simulink model "bpsk_demod_architecture"  (R2023a)
settings: Solver=VariableStepAuto  StartTime=0.0  StopTime=10.0  RelTol=1e-3
settings Model: DataDictionary=bpsk_demod_interfaces.sldd  Creator=kaichiota  LastModifiedBy=kaichiota

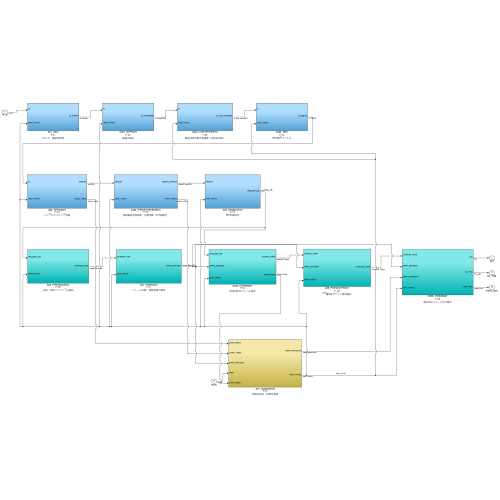
[thumbnail: Simulink's stored preview of the top-level diagram]
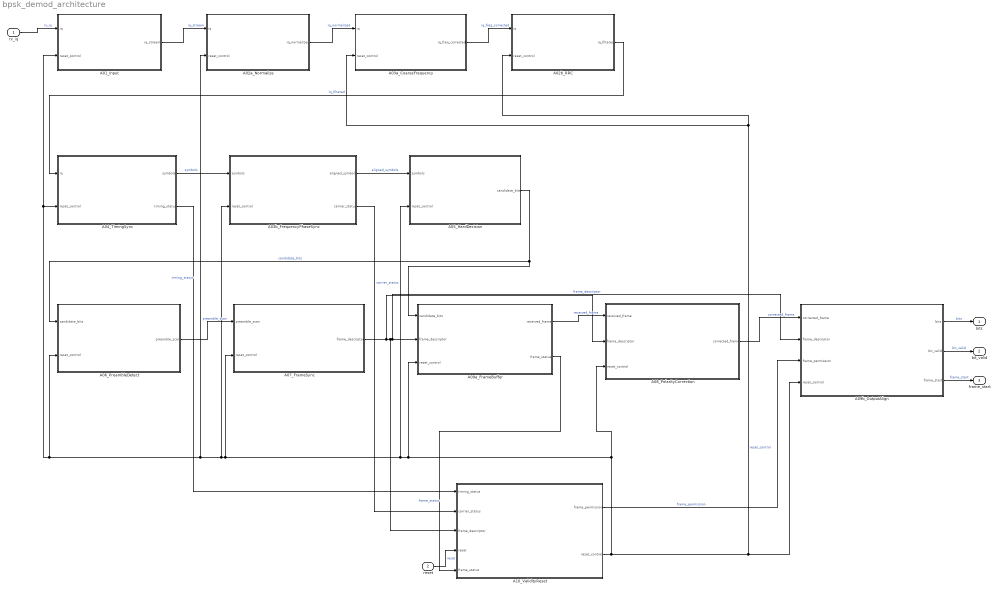
== system bpsk_demod_architecture ==
  rx_iq : Inport  Description=|  OutDataTypeStr=double  PortDimensions=1
      | IF-01 | rx_iq | complex double
      | 80 ksample/s。外部resetがfalseの間は連続入力。
      | Reset: reset中は消費しない。外部入力ポートは追加しない。
      settings: SignalType=complex
  reset : Inport  Description=|  Port=2  OutDataTypeStr=boolean  PortDimensions=1
      | IF-16 | reset | boolean
      | true中は初期化保持。
      | Reset: 外部resetを優先。bits/bit_valid/frame_startを0/false/falseへ。
  A01_Input : Subsystem  Description=|
      | F-01: IQ入力・連続性管理
      | Static architecture only. Inport/Outport placeholders; no executable algorithm. Logical signals carry position/validity metadata; data types, sizes and sample times are not specified.
      settings: AttributesFormatString=|
      | F-01
      | IQ入力・連続性管理
  A02a_Normalize : Subsystem  Description=|
      | F-02: 振幅正規化
      | Static architecture only. Inport/Outport placeholders; no executable algorithm. Logical signals carry position/validity metadata; data types, sizes and sample times are not specified.
      settings: AttributesFormatString=|
      | F-02
      | 振幅正規化
  A02b_RRC : Subsystem  Description=|
      | F-02: RRC整合フィルタ
      | Static architecture only. Inport/Outport placeholders; no executable algorithm. Logical signals carry position/validity metadata; data types, sizes and sample times are not specified.
      settings: AttributesFormatString=|
      | F-02
      | RRC整合フィルタ
  A03a_CoarseFrequency : Subsystem  Description=|
      | F-03: 搬送波周波数の粗補償（位相未同期）
      | Static architecture only. Inport/Outport placeholders; no executable algorithm. Logical signals carry position/validity metadata; data types, sizes and sample times are not specified.
      settings: AttributesFormatString=|
      | F-03
      | 搬送波周波数の粗補償（位相未同期）
  A03b_FrequencyPhaseSync : Subsystem  Description=|
      | F-03: 残留搬送波周波数・位相同期（0/π未確定）
      | Static architecture only. Inport/Outport placeholders; no executable algorithm. Logical signals carry position/validity metadata; data types, sizes and sample times are not specified.
      settings: AttributesFormatString=|
      | F-03
      | 残留搬送波周波数・位相同期（0/π未確定）
  A04_TimingSync : Subsystem  Description=|
      | F-04: シンボルタイミング同期
      | Static architecture only. Inport/Outport placeholders; no executable algorithm. Logical signals carry position/validity metadata; data types, sizes and sample times are not specified.
      settings: AttributesFormatString=|
      | F-04
      | シンボルタイミング同期
  A05_HardDecision : Subsystem  Description=|
      | F-05: BPSK硬判定
      | Static architecture only. Inport/Outport placeholders; no executable algorithm. Logical signals carry position/validity metadata; data types, sizes and sample times are not specified.
      settings: AttributesFormatString=|
      | F-05
      | BPSK硬判定
  A06_PreambleDetect : Subsystem  Description=|
      | F-06: 正規・反転プリアンブル識別
      | Static architecture only. Inport/Outport placeholders; no executable algorithm. Logical signals carry position/validity metadata; data types, sizes and sample times are not specified.
      settings: AttributesFormatString=|
      | F-06
      | 正規・反転プリアンブル識別
  A07_FrameSync : Subsystem  Description=|
      | F-07: フレーム位置・極性情報の確定
      | Static architecture only. Inport/Outport placeholders; no executable algorithm. Logical signals carry position/validity metadata; data types, sizes and sample times are not specified.
      settings: AttributesFormatString=|
      | F-07
      | フレーム位置・極性情報の確定
  A08_PolarityCorrection : Subsystem  Description=|
      | F-08: 0/π曖昧性のビット極性補正
      | Static architecture only. Inport/Outport placeholders; no executable algorithm. Logical signals carry position/validity metadata; data types, sizes and sample times are not specified.
      settings: AttributesFormatString=|
      | F-08
      | 0/π曖昧性のビット極性補正
  A09a_FrameBuffer : Subsystem  Description=|
      | F-09: 受信288 bitフレーム保持
      | Static architecture only. Inport/Outport placeholders; no executable algorithm. Logical signals carry position/validity metadata; data types, sizes and sample times are not specified.
      settings: AttributesFormatString=|
      | F-09
      | 受信288 bitフレーム保持
  A09b_OutputAlign : Subsystem  Description=|
      | F-09: 補正済みフレーム出力整列
      | Static architecture only. Inport/Outport placeholders; no executable algorithm. Logical signals carry position/validity metadata; data types, sizes and sample times are not specified.
      settings: AttributesFormatString=|
      | F-09
      | 補正済みフレーム出力整列
  A10_ValidityReset : Subsystem  Description=|
      | F-10: 同期有効性・初期化管理
      | Static architecture only. Inport/Outport placeholders; no executable algorithm. Logical signals carry position/validity metadata; data types, sizes and sample times are not specified.
      settings: AttributesFormatString=|
      | F-10
      | 同期有効性・初期化管理
  bits : Outport  Description=|  OutDataTypeStr=uint8  PortDimensions=1
      | IF-18 | bits | uint8
      | 公称10 kbit/s、bit_valid=true時のみ意味を持つ。
      | Reset: reset時0。無効区間も0。
  bit_valid : Outport  Description=|  Port=2  OutDataTypeStr=boolean  PortDimensions=1
      | IF-19 | bit_valid | boolean
      | bitsと同時。同期・位置・極性が確定した対象フレームの送出時にtrue。
      | Reset: reset時false。
  frame_start : Outport  Description=|  Port=3  OutDataTypeStr=boolean  PortDimensions=1
      | IF-20 | frame_start | boolean
      | bit_valid=trueかつフレームの最初のbitのみtrue。
      | Reset: reset時false。
  wires:
  A09b_OutputAlign/3(frame_start) -> frame_start/1  "frame_start"
  A09b_OutputAlign/2(bit_valid) -> bit_valid/1  "bit_valid"
  A09b_OutputAlign/1(bits) -> bits/1  "bits"
  A10_ValidityReset/2(reset_control) -> A03a_CoarseFrequency/2(reset_control), A02b_RRC/2(reset_control), A09b_OutputAlign/4(reset_control), A01_Input/2(reset_control), A04_TimingSync/2(reset_control), A06_PreambleDetect/2(reset_control), A02a_Normalize/2(reset_control), A03b_FrequencyPhaseSync/2(reset_control), A07_FrameSync/2(reset_control), A05_HardDecision/2(reset_control), A09a_FrameBuffer/3(reset_control), A08_PolarityCorrection/3(reset_control)  "reset_control"
  reset/1 -> A10_ValidityReset/4(reset)  "reset"
  A10_ValidityReset/1(frame_permission) -> A09b_OutputAlign/3(frame_permission)  "frame_permission"
  A03b_FrequencyPhaseSync/2(carrier_status) -> A10_ValidityReset/2(carrier_status)  "carrier_status"
  A04_TimingSync/2(timing_status) -> A10_ValidityReset/1(timing_status)  "timing_status"
  A08_PolarityCorrection/1(corrected_frame) -> A09b_OutputAlign/1(corrected_frame)  "corrected_frame"
  A09a_FrameBuffer/1(received_frame) -> A08_PolarityCorrection/1(received_frame)  "received_frame"
  A07_FrameSync/1(frame_descriptor) -> A09b_OutputAlign/2(frame_descriptor), A09a_FrameBuffer/2(frame_descriptor), A10_ValidityReset/3(frame_descriptor), A08_PolarityCorrection/2(frame_descriptor)  "frame_descriptor"
  A06_PreambleDetect/1(preamble_scan) -> A07_FrameSync/1(preamble_scan)  "preamble_scan"
  A05_HardDecision/1(candidate_bits) -> A09a_FrameBuffer/1(candidate_bits), A06_PreambleDetect/1(candidate_bits)  "candidate_bits"
  A03b_FrequencyPhaseSync/1(aligned_symbols) -> A05_HardDecision/1(symbols)  "aligned_symbols"
  A04_TimingSync/1(symbols) -> A03b_FrequencyPhaseSync/1(symbols)  "symbols"
  A02b_RRC/1(iq_filtered) -> A04_TimingSync/1(iq)  "iq_filtered"
  A03a_CoarseFrequency/1(iq_freq_corrected) -> A02b_RRC/1(iq)  "iq_freq_corrected"
  A02a_Normalize/1(iq_normalized) -> A03a_CoarseFrequency/1(iq)  "iq_normalized"
  A01_Input/1(iq_stream) -> A02a_Normalize/1(iq)  "iq_stream"
  rx_iq/1 -> A01_Input/1(iq)  "rx_iq"
  A09a_FrameBuffer/2(frame_status) -> A10_ValidityReset/5(frame_status)  "frame_status"

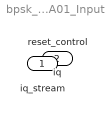
== system bpsk_demod_architecture/A01_Input ==
  iq : Inport  Description=|  OutDataTypeStr=double  PortDimensions=1
      | IF-01 | rx_iq | complex double
      | 80 ksample/s。外部resetがfalseの間は連続入力。
      | Reset: reset中は消費しない。外部入力ポートは追加しない。
      settings: SignalType=complex
  reset_control : Inport  Description=|  Port=2  OutDataTypeStr=Bus: ResetControl
      | IF-17 | reset_control | ResetControl
      | データより先に適用。resetは全初期化、epoch更新のみは再捕捉。
      | Reset: 外部reset区間の開始または再捕捉要求ごとにepochを1回更新。reset保持中は維持。再捕捉時はA-09b受理済みの許可済み完成フレームを保持し、外部resetでは全破棄。
      | reset: boolean scalar — trueの間は保持状態・出力有効を初期化し新規データを消費しない。
      | epoch: uint64 scalar — 実行開始は0。外部reset区間の開始または再捕捉要求ごとに更新し、reset保持中は維持。reset=falseでの更新は再捕捉。旧epochの未許可情報を破棄し、A-09bで受理済みの許可済み完成フレームだけ送出を継続する。
  iq_stream : Outport  Description=|  OutDataTypeStr=Bus: IqRecord
      | IF-02 | iq_stream | IqRecord
      | 80 ksample/s、valid時のみ消費。
      | Reset: 初期化時はvalid=false、旧epochの情報を破棄。
      | valid: boolean scalar — 新しいレコードがある場合true。false時は他フィールドを消費しない。
      | epoch: uint64 scalar — 初期化区間のID。異なるepochのデータ・制御を結合しない。
      | sample_index: uint64 scalar — A-01が付与する0始まり入力サンプル位置。80 ksample/s処理間で維持。
      | value: complex double scalar — 受信または処理後IQ。
      | usable: boolean scalar — 後続の同期判定への利用可否。A-03aは入力の利用可否と粗周波数推定の利用可否を反映し、A-02bはフィルタ過渡も加味する。falseは後段でtrueに上書きしない。具体判定条件は次工程。

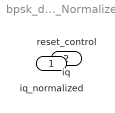
== system bpsk_demod_architecture/A02a_Normalize ==
  iq : Inport  Description=|  OutDataTypeStr=Bus: IqRecord
      | IF-02 | iq_stream | IqRecord
      | 80 ksample/s、valid時のみ消費。
      | Reset: 初期化時はvalid=false、旧epochの情報を破棄。
      | valid: boolean scalar — 新しいレコードがある場合true。false時は他フィールドを消費しない。
      | epoch: uint64 scalar — 初期化区間のID。異なるepochのデータ・制御を結合しない。
      | sample_index: uint64 scalar — A-01が付与する0始まり入力サンプル位置。80 ksample/s処理間で維持。
      | value: complex double scalar — 受信または処理後IQ。
      | usable: boolean scalar — 後続の同期判定への利用可否。A-03aは入力の利用可否と粗周波数推定の利用可否を反映し、A-02bはフィルタ過渡も加味する。falseは後段でtrueに上書きしない。具体判定条件は次工程。
  reset_control : Inport  Description=|  Port=2  OutDataTypeStr=Bus: ResetControl
      | IF-17 | reset_control | ResetControl
      | データより先に適用。resetは全初期化、epoch更新のみは再捕捉。
      | Reset: 外部reset区間の開始または再捕捉要求ごとにepochを1回更新。reset保持中は維持。再捕捉時はA-09b受理済みの許可済み完成フレームを保持し、外部resetでは全破棄。
      | reset: boolean scalar — trueの間は保持状態・出力有効を初期化し新規データを消費しない。
      | epoch: uint64 scalar — 実行開始は0。外部reset区間の開始または再捕捉要求ごとに更新し、reset保持中は維持。reset=falseでの更新は再捕捉。旧epochの未許可情報を破棄し、A-09bで受理済みの許可済み完成フレームだけ送出を継続する。
  iq_normalized : Outport  Description=|  OutDataTypeStr=Bus: IqRecord
      | IF-03 | iq_normalized | IqRecord
      | 80 ksample/s、valid時のみ消費。
      | Reset: 初期化時はvalid=false、旧epochの情報を破棄。
      | valid: boolean scalar — 新しいレコードがある場合true。false時は他フィールドを消費しない。
      | epoch: uint64 scalar — 初期化区間のID。異なるepochのデータ・制御を結合しない。
      | sample_index: uint64 scalar — A-01が付与する0始まり入力サンプル位置。80 ksample/s処理間で維持。
      | value: complex double scalar — 受信または処理後IQ。
      | usable: boolean scalar — 後続の同期判定への利用可否。A-03aは入力の利用可否と粗周波数推定の利用可否を反映し、A-02bはフィルタ過渡も加味する。falseは後段でtrueに上書きしない。具体判定条件は次工程。

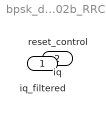
== system bpsk_demod_architecture/A02b_RRC ==
  iq : Inport  Description=|  OutDataTypeStr=Bus: IqRecord
      | IF-04 | iq_freq_corrected | IqRecord
      | 80 ksample/s、valid時のみ消費。
      | Reset: 初期化時はvalid=false、旧epochの情報を破棄。
      | valid: boolean scalar — 新しいレコードがある場合true。false時は他フィールドを消費しない。
      | epoch: uint64 scalar — 初期化区間のID。異なるepochのデータ・制御を結合しない。
      | sample_index: uint64 scalar — A-01が付与する0始まり入力サンプル位置。80 ksample/s処理間で維持。
      | value: complex double scalar — 受信または処理後IQ。
      | usable: boolean scalar — 後続の同期判定への利用可否。A-03aは入力の利用可否と粗周波数推定の利用可否を反映し、A-02bはフィルタ過渡も加味する。falseは後段でtrueに上書きしない。具体判定条件は次工程。
  reset_control : Inport  Description=|  Port=2  OutDataTypeStr=Bus: ResetControl
      | IF-17 | reset_control | ResetControl
      | データより先に適用。resetは全初期化、epoch更新のみは再捕捉。
      | Reset: 外部reset区間の開始または再捕捉要求ごとにepochを1回更新。reset保持中は維持。再捕捉時はA-09b受理済みの許可済み完成フレームを保持し、外部resetでは全破棄。
      | reset: boolean scalar — trueの間は保持状態・出力有効を初期化し新規データを消費しない。
      | epoch: uint64 scalar — 実行開始は0。外部reset区間の開始または再捕捉要求ごとに更新し、reset保持中は維持。reset=falseでの更新は再捕捉。旧epochの未許可情報を破棄し、A-09bで受理済みの許可済み完成フレームだけ送出を継続する。
  iq_filtered : Outport  Description=|  OutDataTypeStr=Bus: IqRecord
      | IF-05 | iq_filtered | IqRecord
      | 80 ksample/s、valid時のみ消費。
      | Reset: 初期化時はvalid=false、旧epochの情報を破棄。
      | valid: boolean scalar — 新しいレコードがある場合true。false時は他フィールドを消費しない。
      | epoch: uint64 scalar — 初期化区間のID。異なるepochのデータ・制御を結合しない。
      | sample_index: uint64 scalar — A-01が付与する0始まり入力サンプル位置。80 ksample/s処理間で維持。
      | value: complex double scalar — 受信または処理後IQ。
      | usable: boolean scalar — 後続の同期判定への利用可否。A-03aは入力の利用可否と粗周波数推定の利用可否を反映し、A-02bはフィルタ過渡も加味する。falseは後段でtrueに上書きしない。具体判定条件は次工程。

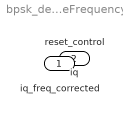
== system bpsk_demod_architecture/A03a_CoarseFrequency ==
  iq : Inport  Description=|  OutDataTypeStr=Bus: IqRecord
      | IF-03 | iq_normalized | IqRecord
      | 80 ksample/s、valid時のみ消費。
      | Reset: 初期化時はvalid=false、旧epochの情報を破棄。
      | valid: boolean scalar — 新しいレコードがある場合true。false時は他フィールドを消費しない。
      | epoch: uint64 scalar — 初期化区間のID。異なるepochのデータ・制御を結合しない。
      | sample_index: uint64 scalar — A-01が付与する0始まり入力サンプル位置。80 ksample/s処理間で維持。
      | value: complex double scalar — 受信または処理後IQ。
      | usable: boolean scalar — 後続の同期判定への利用可否。A-03aは入力の利用可否と粗周波数推定の利用可否を反映し、A-02bはフィルタ過渡も加味する。falseは後段でtrueに上書きしない。具体判定条件は次工程。
  reset_control : Inport  Description=|  Port=2  OutDataTypeStr=Bus: ResetControl
      | IF-17 | reset_control | ResetControl
      | データより先に適用。resetは全初期化、epoch更新のみは再捕捉。
      | Reset: 外部reset区間の開始または再捕捉要求ごとにepochを1回更新。reset保持中は維持。再捕捉時はA-09b受理済みの許可済み完成フレームを保持し、外部resetでは全破棄。
      | reset: boolean scalar — trueの間は保持状態・出力有効を初期化し新規データを消費しない。
      | epoch: uint64 scalar — 実行開始は0。外部reset区間の開始または再捕捉要求ごとに更新し、reset保持中は維持。reset=falseでの更新は再捕捉。旧epochの未許可情報を破棄し、A-09bで受理済みの許可済み完成フレームだけ送出を継続する。
  iq_freq_corrected : Outport  Description=|  OutDataTypeStr=Bus: IqRecord
      | IF-04 | iq_freq_corrected | IqRecord
      | 80 ksample/s、valid時のみ消費。
      | Reset: 初期化時はvalid=false、旧epochの情報を破棄。
      | valid: boolean scalar — 新しいレコードがある場合true。false時は他フィールドを消費しない。
      | epoch: uint64 scalar — 初期化区間のID。異なるepochのデータ・制御を結合しない。
      | sample_index: uint64 scalar — A-01が付与する0始まり入力サンプル位置。80 ksample/s処理間で維持。
      | value: complex double scalar — 受信または処理後IQ。
      | usable: boolean scalar — 後続の同期判定への利用可否。A-03aは入力の利用可否と粗周波数推定の利用可否を反映し、A-02bはフィルタ過渡も加味する。falseは後段でtrueに上書きしない。具体判定条件は次工程。

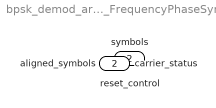
== system bpsk_demod_architecture/A03b_FrequencyPhaseSync ==
  symbols : Inport  Description=|  OutDataTypeStr=Bus: SymbolRecord
      | IF-06 | symbols | SymbolRecord
      | 公称10 ksymbol/s。validな候補ごとに更新。
      | Reset: 初期化時はvalid=false、旧epochの情報を破棄。
      | valid: boolean scalar — 新しいレコードがある場合true。false時は他フィールドを消費しない。
      | epoch: uint64 scalar — 初期化区間のID。異なるepochのデータ・制御を結合しない。
      | symbol_index: uint64 scalar — A-04が候補シンボル生成順に0から付与。同期未確立でも生成した候補は数える。
      | value: complex double scalar — 抽出または搬送波補償後のシンボル。
      | timing_locked: boolean scalar — 当該シンボルに対応するタイミング同期状態。入力usableも加味する。
      | carrier_locked: boolean scalar — 当該シンボルの搬送波同期状態。A-04ではfalse、A-03bが設定。
  reset_control : Inport  Description=|  Port=2  OutDataTypeStr=Bus: ResetControl
      | IF-17 | reset_control | ResetControl
      | データより先に適用。resetは全初期化、epoch更新のみは再捕捉。
      | Reset: 外部reset区間の開始または再捕捉要求ごとにepochを1回更新。reset保持中は維持。再捕捉時はA-09b受理済みの許可済み完成フレームを保持し、外部resetでは全破棄。
      | reset: boolean scalar — trueの間は保持状態・出力有効を初期化し新規データを消費しない。
      | epoch: uint64 scalar — 実行開始は0。外部reset区間の開始または再捕捉要求ごとに更新し、reset保持中は維持。reset=falseでの更新は再捕捉。旧epochの未許可情報を破棄し、A-09bで受理済みの許可済み完成フレームだけ送出を継続する。
  aligned_symbols : Outport  Description=|  OutDataTypeStr=Bus: SymbolRecord
      | IF-07 | aligned_symbols | SymbolRecord
      | IF-06の位置を保持。
      | Reset: 初期化時はvalid=false、旧epochの情報を破棄。
      | valid: boolean scalar — 新しいレコードがある場合true。false時は他フィールドを消費しない。
      | epoch: uint64 scalar — 初期化区間のID。異なるepochのデータ・制御を結合しない。
      | symbol_index: uint64 scalar — A-04が候補シンボル生成順に0から付与。同期未確立でも生成した候補は数える。
      | value: complex double scalar — 抽出または搬送波補償後のシンボル。
      | timing_locked: boolean scalar — 当該シンボルに対応するタイミング同期状態。入力usableも加味する。
      | carrier_locked: boolean scalar — 当該シンボルの搬送波同期状態。A-04ではfalse、A-03bが設定。
  carrier_status : Outport  Description=|  Port=2  OutDataTypeStr=Bus: SyncStatus
      | IF-14 | carrier_status | SyncStatus
      | 候補シンボルごとの搬送波同期状態。
      | Reset: 初期化時はvalid=false、旧epochの情報を破棄。
      | valid: boolean scalar — 新しいレコードがある場合true。false時は他フィールドを消費しない。
      | epoch: uint64 scalar — 初期化区間のID。異なるepochのデータ・制御を結合しない。
      | symbol_index: uint64 scalar — この同期判定が対応する候補シンボル位置。
      | locked: boolean scalar — タイミングまたは搬送波の同期成立判定。具体閾値・継続条件は次工程。

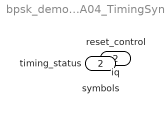
== system bpsk_demod_architecture/A04_TimingSync ==
  iq : Inport  Description=|  OutDataTypeStr=Bus: IqRecord
      | IF-05 | iq_filtered | IqRecord
      | 80 ksample/s、valid時のみ消費。
      | Reset: 初期化時はvalid=false、旧epochの情報を破棄。
      | valid: boolean scalar — 新しいレコードがある場合true。false時は他フィールドを消費しない。
      | epoch: uint64 scalar — 初期化区間のID。異なるepochのデータ・制御を結合しない。
      | sample_index: uint64 scalar — A-01が付与する0始まり入力サンプル位置。80 ksample/s処理間で維持。
      | value: complex double scalar — 受信または処理後IQ。
      | usable: boolean scalar — 後続の同期判定への利用可否。A-03aは入力の利用可否と粗周波数推定の利用可否を反映し、A-02bはフィルタ過渡も加味する。falseは後段でtrueに上書きしない。具体判定条件は次工程。
  reset_control : Inport  Description=|  Port=2  OutDataTypeStr=Bus: ResetControl
      | IF-17 | reset_control | ResetControl
      | データより先に適用。resetは全初期化、epoch更新のみは再捕捉。
      | Reset: 外部reset区間の開始または再捕捉要求ごとにepochを1回更新。reset保持中は維持。再捕捉時はA-09b受理済みの許可済み完成フレームを保持し、外部resetでは全破棄。
      | reset: boolean scalar — trueの間は保持状態・出力有効を初期化し新規データを消費しない。
      | epoch: uint64 scalar — 実行開始は0。外部reset区間の開始または再捕捉要求ごとに更新し、reset保持中は維持。reset=falseでの更新は再捕捉。旧epochの未許可情報を破棄し、A-09bで受理済みの許可済み完成フレームだけ送出を継続する。
  symbols : Outport  Description=|  OutDataTypeStr=Bus: SymbolRecord
      | IF-06 | symbols | SymbolRecord
      | 公称10 ksymbol/s。validな候補ごとに更新。
      | Reset: 初期化時はvalid=false、旧epochの情報を破棄。
      | valid: boolean scalar — 新しいレコードがある場合true。false時は他フィールドを消費しない。
      | epoch: uint64 scalar — 初期化区間のID。異なるepochのデータ・制御を結合しない。
      | symbol_index: uint64 scalar — A-04が候補シンボル生成順に0から付与。同期未確立でも生成した候補は数える。
      | value: complex double scalar — 抽出または搬送波補償後のシンボル。
      | timing_locked: boolean scalar — 当該シンボルに対応するタイミング同期状態。入力usableも加味する。
      | carrier_locked: boolean scalar — 当該シンボルの搬送波同期状態。A-04ではfalse、A-03bが設定。
  timing_status : Outport  Description=|  Port=2  OutDataTypeStr=Bus: SyncStatus
      | IF-13 | timing_status | SyncStatus
      | 候補シンボルごとのタイミング同期状態。
      | Reset: 初期化時はvalid=false、旧epochの情報を破棄。
      | valid: boolean scalar — 新しいレコードがある場合true。false時は他フィールドを消費しない。
      | epoch: uint64 scalar — 初期化区間のID。異なるepochのデータ・制御を結合しない。
      | symbol_index: uint64 scalar — この同期判定が対応する候補シンボル位置。
      | locked: boolean scalar — タイミングまたは搬送波の同期成立判定。具体閾値・継続条件は次工程。

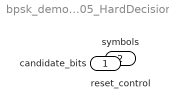
== system bpsk_demod_architecture/A05_HardDecision ==
  symbols : Inport  Description=|  OutDataTypeStr=Bus: SymbolRecord
      | IF-07 | aligned_symbols | SymbolRecord
      | IF-06の位置を保持。
      | Reset: 初期化時はvalid=false、旧epochの情報を破棄。
      | valid: boolean scalar — 新しいレコードがある場合true。false時は他フィールドを消費しない。
      | epoch: uint64 scalar — 初期化区間のID。異なるepochのデータ・制御を結合しない。
      | symbol_index: uint64 scalar — A-04が候補シンボル生成順に0から付与。同期未確立でも生成した候補は数える。
      | value: complex double scalar — 抽出または搬送波補償後のシンボル。
      | timing_locked: boolean scalar — 当該シンボルに対応するタイミング同期状態。入力usableも加味する。
      | carrier_locked: boolean scalar — 当該シンボルの搬送波同期状態。A-04ではfalse、A-03bが設定。
  reset_control : Inport  Description=|  Port=2  OutDataTypeStr=Bus: ResetControl
      | IF-17 | reset_control | ResetControl
      | データより先に適用。resetは全初期化、epoch更新のみは再捕捉。
      | Reset: 外部reset区間の開始または再捕捉要求ごとにepochを1回更新。reset保持中は維持。再捕捉時はA-09b受理済みの許可済み完成フレームを保持し、外部resetでは全破棄。
      | reset: boolean scalar — trueの間は保持状態・出力有効を初期化し新規データを消費しない。
      | epoch: uint64 scalar — 実行開始は0。外部reset区間の開始または再捕捉要求ごとに更新し、reset保持中は維持。reset=falseでの更新は再捕捉。旧epochの未許可情報を破棄し、A-09bで受理済みの許可済み完成フレームだけ送出を継続する。
  candidate_bits : Outport  Description=|  OutDataTypeStr=Bus: BitRecord
      | IF-08 | candidate_bits | BitRecord
      | 公称10 kbit/s。validとsync_okを区別。
      | Reset: 初期化時はvalid=false、旧epochの情報を破棄。
      | valid: boolean scalar — 新しいレコードがある場合true。false時は他フィールドを消費しない。
      | epoch: uint64 scalar — 初期化区間のID。異なるepochのデータ・制御を結合しない。
      | bit_index: uint64 scalar — 対応するsymbol_indexをそのまま継承。候補bitの0始まり位置。
      | value: uint8 scalar — 極性未確定の硬判定0/1。
      | sync_ok: boolean scalar — 当該シンボルのtiming_locked AND carrier_locked。falseでもvalidな候補は位置を進める。

== system bpsk_demod_architecture/A06_PreambleDetect ==
  candidate_bits : Inport  Description=|  OutDataTypeStr=Bus: BitRecord
      | IF-08 | candidate_bits | BitRecord
      | 公称10 kbit/s。validとsync_okを区別。
      | Reset: 初期化時はvalid=false、旧epochの情報を破棄。
      | valid: boolean scalar — 新しいレコードがある場合true。false時は他フィールドを消費しない。
      | epoch: uint64 scalar — 初期化区間のID。異なるepochのデータ・制御を結合しない。
      | bit_index: uint64 scalar — 対応するsymbol_indexをそのまま継承。候補bitの0始まり位置。
      | value: uint8 scalar — 極性未確定の硬判定0/1。
      | sync_ok: boolean scalar — 当該シンボルのtiming_locked AND carrier_locked。falseでもvalidな候補は位置を進める。
  reset_control : Inport  Description=|  Port=2  OutDataTypeStr=Bus: ResetControl
      | IF-17 | reset_control | ResetControl
      | データより先に適用。resetは全初期化、epoch更新のみは再捕捉。
      | Reset: 外部reset区間の開始または再捕捉要求ごとにepochを1回更新。reset保持中は維持。再捕捉時はA-09b受理済みの許可済み完成フレームを保持し、外部resetでは全破棄。
      | reset: boolean scalar — trueの間は保持状態・出力有効を初期化し新規データを消費しない。
      | epoch: uint64 scalar — 実行開始は0。外部reset区間の開始または再捕捉要求ごとに更新し、reset保持中は維持。reset=falseでの更新は再捕捉。旧epochの未許可情報を破棄し、A-09bで受理済みの許可済み完成フレームだけ送出を継続する。
  preamble_scan : Outport  Description=|  OutDataTypeStr=Bus: PreambleScan
      | IF-09 | preamble_scan | PreambleScan
      | 候補bitごと。未検出時もvalid=trueで進捗を通知。
      | Reset: 初期化時はvalid=false、旧epochの情報を破棄。
      | valid: boolean scalar — 新しいレコードがある場合true。false時は他フィールドを消費しない。
      | epoch: uint64 scalar — 初期化区間のID。異なるepochのデータ・制御を結合しない。
      | bit_index: uint64 scalar — 照合窓末尾の候補bit位置。未検出時も通知し、A-07が期待位置を通過したことを認識できる。
      | window_ready: boolean scalar — 連続した32 bitの窓が揃ったか。
      | match_found: boolean scalar — 正規または反転パターンの候補として採用可能か。閾値・同点処理は未定。
      | start_bit: uint64 scalar — window_ready時のみ有効。bit_index-31。
      | invert: boolean scalar — match_found時のみ有効。trueなら全bit反転候補。
      | errors_normal: uint8 scalar — window_ready時の正規プリアンブルとの不一致数0〜32。
      | errors_inverted: uint8 scalar — window_ready時の反転プリアンブルとの不一致数0〜32。
      | window_sync_ok: boolean scalar — 照合対象32 bitすべてでsync_okがtrueか。

== system bpsk_demod_architecture/A07_FrameSync ==
  preamble_scan : Inport  Description=|  OutDataTypeStr=Bus: PreambleScan
      | IF-09 | preamble_scan | PreambleScan
      | 候補bitごと。未検出時もvalid=trueで進捗を通知。
      | Reset: 初期化時はvalid=false、旧epochの情報を破棄。
      | valid: boolean scalar — 新しいレコードがある場合true。false時は他フィールドを消費しない。
      | epoch: uint64 scalar — 初期化区間のID。異なるepochのデータ・制御を結合しない。
      | bit_index: uint64 scalar — 照合窓末尾の候補bit位置。未検出時も通知し、A-07が期待位置を通過したことを認識できる。
      | window_ready: boolean scalar — 連続した32 bitの窓が揃ったか。
      | match_found: boolean scalar — 正規または反転パターンの候補として採用可能か。閾値・同点処理は未定。
      | start_bit: uint64 scalar — window_ready時のみ有効。bit_index-31。
      | invert: boolean scalar — match_found時のみ有効。trueなら全bit反転候補。
      | errors_normal: uint8 scalar — window_ready時の正規プリアンブルとの不一致数0〜32。
      | errors_inverted: uint8 scalar — window_ready時の反転プリアンブルとの不一致数0〜32。
      | window_sync_ok: boolean scalar — 照合対象32 bitすべてでsync_okがtrueか。
  reset_control : Inport  Description=|  Port=2  OutDataTypeStr=Bus: ResetControl
      | IF-17 | reset_control | ResetControl
      | データより先に適用。resetは全初期化、epoch更新のみは再捕捉。
      | Reset: 外部reset区間の開始または再捕捉要求ごとにepochを1回更新。reset保持中は維持。再捕捉時はA-09b受理済みの許可済み完成フレームを保持し、外部resetでは全破棄。
      | reset: boolean scalar — trueの間は保持状態・出力有効を初期化し新規データを消費しない。
      | epoch: uint64 scalar — 実行開始は0。外部reset区間の開始または再捕捉要求ごとに更新し、reset保持中は維持。reset=falseでの更新は再捕捉。旧epochの未許可情報を破棄し、A-09bで受理済みの許可済み完成フレームだけ送出を継続する。
  frame_descriptor : Outport  Description=|  OutDataTypeStr=Bus: FrameDescriptor
      | IF-10 | frame_descriptor | FrameDescriptor
      | フレーム判断イベント。位置・極性が揃うまでconfirmed=false。
      | Reset: 初期化時はvalid=false、旧epochの情報を破棄。
      | valid: boolean scalar — 新しいレコードがある場合true。false時は他フィールドを消費しない。
      | epoch: uint64 scalar — 初期化区間のID。異なるepochのデータ・制御を結合しない。
      | start_bit: uint64 scalar — 対象フレームのプリアンブル先頭bit位置。epochと合わせてフレームキーとする。
      | confirmed: boolean scalar — 当該フレームの位置とプリアンブルが確認済みか。未検出等ではfalse。
      | polarity_valid: boolean scalar — invertが有効な極性判断か。
      | invert: boolean scalar — trueなら対象288 bitを反転。polarity_valid=falseのとき解釈しない。

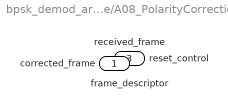
== system bpsk_demod_architecture/A08_PolarityCorrection ==
  received_frame : Inport  Description=|  OutDataTypeStr=Bus: ReceivedFrame
      | IF-11 | received_frame | ReceivedFrame
      | 完成フレームごと。未完成のbit配列は出さない。
      | Reset: 初期化時はvalid=false、旧epochの情報を破棄。
      | valid: boolean scalar — 新しいレコードがある場合true。false時は他フィールドを消費しない。
      | epoch: uint64 scalar — 初期化区間のID。異なるepochのデータ・制御を結合しない。
      | start_bit: uint64 scalar — 保持フレームの先頭。
      | bits: uint8 [288,1] — 受信順の0/1。先頭32要素がプリアンブル、残り256要素がデータ。
      | sync_ok_all: boolean scalar — 対象288 bitのsync_okの論理積。現在のロック状態で代用しない。
  frame_descriptor : Inport  Description=|  Port=2  OutDataTypeStr=Bus: FrameDescriptor
      | IF-10 | frame_descriptor | FrameDescriptor
      | フレーム判断イベント。位置・極性が揃うまでconfirmed=false。
      | Reset: 初期化時はvalid=false、旧epochの情報を破棄。
      | valid: boolean scalar — 新しいレコードがある場合true。false時は他フィールドを消費しない。
      | epoch: uint64 scalar — 初期化区間のID。異なるepochのデータ・制御を結合しない。
      | start_bit: uint64 scalar — 対象フレームのプリアンブル先頭bit位置。epochと合わせてフレームキーとする。
      | confirmed: boolean scalar — 当該フレームの位置とプリアンブルが確認済みか。未検出等ではfalse。
      | polarity_valid: boolean scalar — invertが有効な極性判断か。
      | invert: boolean scalar — trueなら対象288 bitを反転。polarity_valid=falseのとき解釈しない。
  reset_control : Inport  Description=|  Port=3  OutDataTypeStr=Bus: ResetControl
      | IF-17 | reset_control | ResetControl
      | データより先に適用。resetは全初期化、epoch更新のみは再捕捉。
      | Reset: 外部reset区間の開始または再捕捉要求ごとにepochを1回更新。reset保持中は維持。再捕捉時はA-09b受理済みの許可済み完成フレームを保持し、外部resetでは全破棄。
      | reset: boolean scalar — trueの間は保持状態・出力有効を初期化し新規データを消費しない。
      | epoch: uint64 scalar — 実行開始は0。外部reset区間の開始または再捕捉要求ごとに更新し、reset保持中は維持。reset=falseでの更新は再捕捉。旧epochの未許可情報を破棄し、A-09bで受理済みの許可済み完成フレームだけ送出を継続する。
  corrected_frame : Outport  Description=|  OutDataTypeStr=Bus: CorrectedFrame
      | IF-12 | corrected_frame | CorrectedFrame
      | 同一キーのReceivedFrameと有効なFrameDescriptorが揃ったとき。
      | Reset: 初期化時はvalid=false、旧epochの情報を破棄。
      | valid: boolean scalar — 新しいレコードがある場合true。false時は他フィールドを消費しない。
      | epoch: uint64 scalar — 初期化区間のID。異なるepochのデータ・制御を結合しない。
      | start_bit: uint64 scalar — 元の受信フレームと同じ先頭。
      | bits: uint8 [288,1] — 極性補正済み0/1。受信プリアンブルも同じ規則で補正し置換しない。
      | sync_ok_all: boolean scalar — ReceivedFrameから継承する。
      | inverted: boolean scalar — 実際に全bit反転を適用したか。

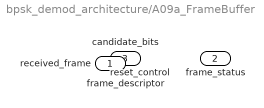
== system bpsk_demod_architecture/A09a_FrameBuffer ==
  candidate_bits : Inport  Description=|  OutDataTypeStr=Bus: BitRecord
      | IF-08 | candidate_bits | BitRecord
      | 公称10 kbit/s。validとsync_okを区別。
      | Reset: 初期化時はvalid=false、旧epochの情報を破棄。
      | valid: boolean scalar — 新しいレコードがある場合true。false時は他フィールドを消費しない。
      | epoch: uint64 scalar — 初期化区間のID。異なるepochのデータ・制御を結合しない。
      | bit_index: uint64 scalar — 対応するsymbol_indexをそのまま継承。候補bitの0始まり位置。
      | value: uint8 scalar — 極性未確定の硬判定0/1。
      | sync_ok: boolean scalar — 当該シンボルのtiming_locked AND carrier_locked。falseでもvalidな候補は位置を進める。
  frame_descriptor : Inport  Description=|  Port=2  OutDataTypeStr=Bus: FrameDescriptor
      | IF-10 | frame_descriptor | FrameDescriptor
      | フレーム判断イベント。位置・極性が揃うまでconfirmed=false。
      | Reset: 初期化時はvalid=false、旧epochの情報を破棄。
      | valid: boolean scalar — 新しいレコードがある場合true。false時は他フィールドを消費しない。
      | epoch: uint64 scalar — 初期化区間のID。異なるepochのデータ・制御を結合しない。
      | start_bit: uint64 scalar — 対象フレームのプリアンブル先頭bit位置。epochと合わせてフレームキーとする。
      | confirmed: boolean scalar — 当該フレームの位置とプリアンブルが確認済みか。未検出等ではfalse。
      | polarity_valid: boolean scalar — invertが有効な極性判断か。
      | invert: boolean scalar — trueなら対象288 bitを反転。polarity_valid=falseのとき解釈しない。
  reset_control : Inport  Description=|  Port=3  OutDataTypeStr=Bus: ResetControl
      | IF-17 | reset_control | ResetControl
      | データより先に適用。resetは全初期化、epoch更新のみは再捕捉。
      | Reset: 外部reset区間の開始または再捕捉要求ごとにepochを1回更新。reset保持中は維持。再捕捉時はA-09b受理済みの許可済み完成フレームを保持し、外部resetでは全破棄。
      | reset: boolean scalar — trueの間は保持状態・出力有効を初期化し新規データを消費しない。
      | epoch: uint64 scalar — 実行開始は0。外部reset区間の開始または再捕捉要求ごとに更新し、reset保持中は維持。reset=falseでの更新は再捕捉。旧epochの未許可情報を破棄し、A-09bで受理済みの許可済み完成フレームだけ送出を継続する。
  received_frame : Outport  Description=|  OutDataTypeStr=Bus: ReceivedFrame
      | IF-11 | received_frame | ReceivedFrame
      | 完成フレームごと。未完成のbit配列は出さない。
      | Reset: 初期化時はvalid=false、旧epochの情報を破棄。
      | valid: boolean scalar — 新しいレコードがある場合true。false時は他フィールドを消費しない。
      | epoch: uint64 scalar — 初期化区間のID。異なるepochのデータ・制御を結合しない。
      | start_bit: uint64 scalar — 保持フレームの先頭。
      | bits: uint8 [288,1] — 受信順の0/1。先頭32要素がプリアンブル、残り256要素がデータ。
      | sync_ok_all: boolean scalar — 対象288 bitのsync_okの論理積。現在のロック状態で代用しない。
  frame_status : Outport  Description=|  Port=2  OutDataTypeStr=Bus: FrameStatus
      | IF-21 | frame_status | FrameStatus
      | フレーム完了または取得失敗を確定したイベント。受信中の同期状態を集約。
      | Reset: 初期化時はvalid=false、旧epochの情報を破棄。
      | valid: boolean scalar — 新しいレコードがある場合true。false時は他フィールドを消費しない。
      | epoch: uint64 scalar — 初期化区間のID。異なるepochのデータ・制御を結合しない。
      | start_bit: uint64 scalar — 評価対象の先頭。
      | complete: boolean scalar — 288 bitが欠落・重複なく揃ったか。
      | sync_ok_all: boolean scalar — completeなフレームの全bitで同期成立していたか。complete=false時はfalse。

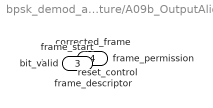
== system bpsk_demod_architecture/A09b_OutputAlign ==
  corrected_frame : Inport  Description=|  OutDataTypeStr=Bus: CorrectedFrame
      | IF-12 | corrected_frame | CorrectedFrame
      | 同一キーのReceivedFrameと有効なFrameDescriptorが揃ったとき。
      | Reset: 初期化時はvalid=false、旧epochの情報を破棄。
      | valid: boolean scalar — 新しいレコードがある場合true。false時は他フィールドを消費しない。
      | epoch: uint64 scalar — 初期化区間のID。異なるepochのデータ・制御を結合しない。
      | start_bit: uint64 scalar — 元の受信フレームと同じ先頭。
      | bits: uint8 [288,1] — 極性補正済み0/1。受信プリアンブルも同じ規則で補正し置換しない。
      | sync_ok_all: boolean scalar — ReceivedFrameから継承する。
      | inverted: boolean scalar — 実際に全bit反転を適用したか。
  frame_descriptor : Inport  Description=|  Port=2  OutDataTypeStr=Bus: FrameDescriptor
      | IF-10 | frame_descriptor | FrameDescriptor
      | フレーム判断イベント。位置・極性が揃うまでconfirmed=false。
      | Reset: 初期化時はvalid=false、旧epochの情報を破棄。
      | valid: boolean scalar — 新しいレコードがある場合true。false時は他フィールドを消費しない。
      | epoch: uint64 scalar — 初期化区間のID。異なるepochのデータ・制御を結合しない。
      | start_bit: uint64 scalar — 対象フレームのプリアンブル先頭bit位置。epochと合わせてフレームキーとする。
      | confirmed: boolean scalar — 当該フレームの位置とプリアンブルが確認済みか。未検出等ではfalse。
      | polarity_valid: boolean scalar — invertが有効な極性判断か。
      | invert: boolean scalar — trueなら対象288 bitを反転。polarity_valid=falseのとき解釈しない。
  frame_permission : Inport  Description=|  Port=3  OutDataTypeStr=Bus: FramePermission
      | IF-15 | frame_permission | FramePermission
      | 対象フレームの完了状態と記述子が揃ったときに判断。
      | Reset: 初期化時はvalid=false、旧epochの情報を破棄。
      | valid: boolean scalar — 新しいレコードがある場合true。false時は他フィールドを消費しない。
      | epoch: uint64 scalar — 初期化区間のID。異なるepochのデータ・制御を結合しない。
      | start_bit: uint64 scalar — 出力判断対象の先頭。
      | allow: boolean scalar — trueなら当該完成フレームの送出を許可。falseなら当該フレームは破棄。
  reset_control : Inport  Description=|  Port=4  OutDataTypeStr=Bus: ResetControl
      | IF-17 | reset_control | ResetControl
      | データより先に適用。resetは全初期化、epoch更新のみは再捕捉。
      | Reset: 外部reset区間の開始または再捕捉要求ごとにepochを1回更新。reset保持中は維持。再捕捉時はA-09b受理済みの許可済み完成フレームを保持し、外部resetでは全破棄。
      | reset: boolean scalar — trueの間は保持状態・出力有効を初期化し新規データを消費しない。
      | epoch: uint64 scalar — 実行開始は0。外部reset区間の開始または再捕捉要求ごとに更新し、reset保持中は維持。reset=falseでの更新は再捕捉。旧epochの未許可情報を破棄し、A-09bで受理済みの許可済み完成フレームだけ送出を継続する。
  bits : Outport  Description=|  OutDataTypeStr=uint8  PortDimensions=1
      | IF-18 | bits | uint8
      | 公称10 kbit/s、bit_valid=true時のみ意味を持つ。
      | Reset: reset時0。無効区間も0。
  bit_valid : Outport  Description=|  Port=2  OutDataTypeStr=boolean  PortDimensions=1
      | IF-19 | bit_valid | boolean
      | bitsと同時。同期・位置・極性が確定した対象フレームの送出時にtrue。
      | Reset: reset時false。
  frame_start : Outport  Description=|  Port=3  OutDataTypeStr=boolean  PortDimensions=1
      | IF-20 | frame_start | boolean
      | bit_valid=trueかつフレームの最初のbitのみtrue。
      | Reset: reset時false。

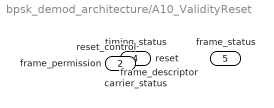
== system bpsk_demod_architecture/A10_ValidityReset ==
  timing_status : Inport  Description=|  OutDataTypeStr=Bus: SyncStatus
      | IF-13 | timing_status | SyncStatus
      | 候補シンボルごとのタイミング同期状態。
      | Reset: 初期化時はvalid=false、旧epochの情報を破棄。
      | valid: boolean scalar — 新しいレコードがある場合true。false時は他フィールドを消費しない。
      | epoch: uint64 scalar — 初期化区間のID。異なるepochのデータ・制御を結合しない。
      | symbol_index: uint64 scalar — この同期判定が対応する候補シンボル位置。
      | locked: boolean scalar — タイミングまたは搬送波の同期成立判定。具体閾値・継続条件は次工程。
  carrier_status : Inport  Description=|  Port=2  OutDataTypeStr=Bus: SyncStatus
      | IF-14 | carrier_status | SyncStatus
      | 候補シンボルごとの搬送波同期状態。
      | Reset: 初期化時はvalid=false、旧epochの情報を破棄。
      | valid: boolean scalar — 新しいレコードがある場合true。false時は他フィールドを消費しない。
      | epoch: uint64 scalar — 初期化区間のID。異なるepochのデータ・制御を結合しない。
      | symbol_index: uint64 scalar — この同期判定が対応する候補シンボル位置。
      | locked: boolean scalar — タイミングまたは搬送波の同期成立判定。具体閾値・継続条件は次工程。
  frame_descriptor : Inport  Description=|  Port=3  OutDataTypeStr=Bus: FrameDescriptor
      | IF-10 | frame_descriptor | FrameDescriptor
      | フレーム判断イベント。位置・極性が揃うまでconfirmed=false。
      | Reset: 初期化時はvalid=false、旧epochの情報を破棄。
      | valid: boolean scalar — 新しいレコードがある場合true。false時は他フィールドを消費しない。
      | epoch: uint64 scalar — 初期化区間のID。異なるepochのデータ・制御を結合しない。
      | start_bit: uint64 scalar — 対象フレームのプリアンブル先頭bit位置。epochと合わせてフレームキーとする。
      | confirmed: boolean scalar — 当該フレームの位置とプリアンブルが確認済みか。未検出等ではfalse。
      | polarity_valid: boolean scalar — invertが有効な極性判断か。
      | invert: boolean scalar — trueなら対象288 bitを反転。polarity_valid=falseのとき解釈しない。
  reset : Inport  Description=|  Port=4  OutDataTypeStr=boolean  PortDimensions=1
      | IF-16 | reset | boolean
      | true中は初期化保持。
      | Reset: 外部resetを優先。bits/bit_valid/frame_startを0/false/falseへ。
  frame_status : Inport  Description=|  Port=5  OutDataTypeStr=Bus: FrameStatus
      | IF-21 | frame_status | FrameStatus
      | フレーム完了または取得失敗を確定したイベント。受信中の同期状態を集約。
      | Reset: 初期化時はvalid=false、旧epochの情報を破棄。
      | valid: boolean scalar — 新しいレコードがある場合true。false時は他フィールドを消費しない。
      | epoch: uint64 scalar — 初期化区間のID。異なるepochのデータ・制御を結合しない。
      | start_bit: uint64 scalar — 評価対象の先頭。
      | complete: boolean scalar — 288 bitが欠落・重複なく揃ったか。
      | sync_ok_all: boolean scalar — completeなフレームの全bitで同期成立していたか。complete=false時はfalse。
  frame_permission : Outport  Description=|  OutDataTypeStr=Bus: FramePermission
      | IF-15 | frame_permission | FramePermission
      | 対象フレームの完了状態と記述子が揃ったときに判断。
      | Reset: 初期化時はvalid=false、旧epochの情報を破棄。
      | valid: boolean scalar — 新しいレコードがある場合true。false時は他フィールドを消費しない。
      | epoch: uint64 scalar — 初期化区間のID。異なるepochのデータ・制御を結合しない。
      | start_bit: uint64 scalar — 出力判断対象の先頭。
      | allow: boolean scalar — trueなら当該完成フレームの送出を許可。falseなら当該フレームは破棄。
  reset_control : Outport  Description=|  Port=2  OutDataTypeStr=Bus: ResetControl
      | IF-17 | reset_control | ResetControl
      | データより先に適用。resetは全初期化、epoch更新のみは再捕捉。
      | Reset: 外部reset区間の開始または再捕捉要求ごとにepochを1回更新。reset保持中は維持。再捕捉時はA-09b受理済みの許可済み完成フレームを保持し、外部resetでは全破棄。
      | reset: boolean scalar — trueの間は保持状態・出力有効を初期化し新規データを消費しない。
      | epoch: uint64 scalar — 実行開始は0。外部reset区間の開始または再捕捉要求ごとに更新し、reset保持中は維持。reset=falseでの更新は再捕捉。旧epochの未許可情報を破棄し、A-09bで受理済みの許可済み完成フレームだけ送出を継続する。
